simulink model "sschdlexTwoLevelConverterIdealModel"  (R2026a)
settings: Solver=FixedStepDiscrete  StopTime=20/fsw  MaxStep=1e-4  RelTol=1e-6  AbsTol=1e-6
InitFcn:
  | ts = 1e-5; % local solver sample period
  | fsw = 1e3; % switching frequency
libraries: nesl_utility x11, ee_lib x7, fl_lib x4, eePwmGeneratorTwoLevel x1
CloseFcn:
  | clear ts fsw;
settings Model: DataTypeOverride=Off  Creator=The MathWorks, Inc.  LastModifiedBy=The MathWorks, Inc.
settings DataIOCC: SaveFormat=StructureWithTime
settings OptimizationCC: ConditionallyExecuteInputs=off  OptimizeBlockIOStorage=off  BufferReuse=off  GlobalBufferReuse=off  ExpressionFolding=off  LocalBlockOutputs=off  OptimizeDataStoreBuffers=off  BusAssignmentInplaceUpdate=off
settings DebuggingCC: AlgebraicLoopMsg=error  SingleTaskRateTransMsg=error  PregeneratedLibrarySubsystemCodeDiagnostic=none
settings HardwareCC: ProdHWDeviceType=ASIC/FPGA->ASIC/FPGA  TargetBitPerLong=64.0  TargetBitPerPointer=64.0  TargetBitPerSizeT=64.0  TargetBitPerPtrDiffT=64.0  TargetLongLongMode=on  TargetIntDivRoundTo=Zero  TargetEndianess=LittleEndian  TargetWordSize=64.0  TargetHWDeviceType=Custom Processor->MATLAB Host Computer  ProdEqTarget=off
settings RTWCC: RTWCompilerOptimization=on
settings SimscapeCC: SimscapeNormalizeSystem=off  SimscapeNominalValues="[{\"value\":\"10\",\"unit\":\"V\"},{\"value\":\"1\",\"unit\":\"A\"},{\"value\":\"10\",\"unit\":\"N*m\"},{\"value\":\"10\",\"unit\":\"bar\"},{\"value\":\"100\",\"unit\":\"kJ/kg\"},{\"value\":\"1\",\"unit\":\"kW\"},{\"value\":\"300\",\"unit\":\"K\"},{\"value\":\"100\",\"unit\":\"cm^3/s\"},{\"value\":\"1\",\"unit\":\"kN\"},{\"value\":\"1\",\"unit\":\"g/cm^3\"},{\"value\":\"1\",\"unit\":\"l\"},{\"value\":\"1\",\"unit\":\"cm^2\"},{\"value\":\"60\",\"unit\":\"Hz\"}]"  SimscapeLogDataHistory=5000.0

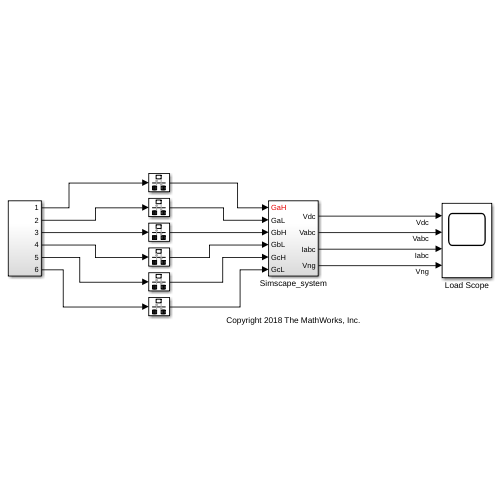
[thumbnail: Simulink's stored preview of the top-level diagram]
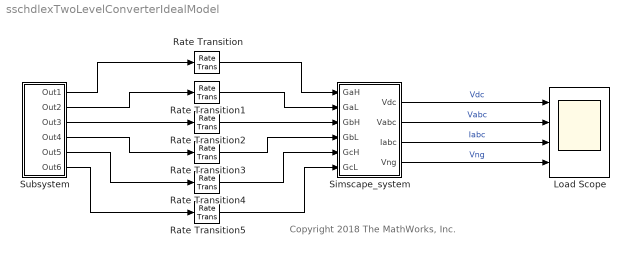
== system sschdlexTwoLevelConverterIdealModel ==
  note: Copyright 2018 The MathWorks, Inc.
  Load Scope : Scope  NumInputPorts=4
      settings: ActiveDisplayYMinimum=300  ActiveDisplayYMaximum=500  DataLoggingSaveFormat=Array
  Rate Transition{,1..5} (6 alike) : RateTransition
  Simscape_system : Subsystem
  Subsystem : Subsystem
  wires:
  Simscape_system/3(Iabc) -> Load Scope/3  "Iabc"
  Simscape_system/1(Vdc) -> Load Scope/1  "Vdc"
  Simscape_system/2(Vabc) -> Load Scope/2  "Vabc"
  Subsystem/1(Out1) -> Rate Transition/1
  Subsystem/2(Out2) -> Rate Transition1/1
  Subsystem/3(Out3) -> Rate Transition2/1
  Subsystem/4(Out4) -> Rate Transition3/1
  Subsystem/5(Out5) -> Rate Transition4/1
  Subsystem/6(Out6) -> Rate Transition5/1
  Rate Transition/1 -> Simscape_system/1(GaH)
  Rate Transition1/1 -> Simscape_system/2(GaL)
  Rate Transition2/1 -> Simscape_system/3(GbH)
  Rate Transition3/1 -> Simscape_system/4(GbL)
  Rate Transition4/1 -> Simscape_system/5(GcH)
  Rate Transition5/1 -> Simscape_system/6(GcL)
  Simscape_system/4(Vng) -> Load Scope/4  "Vng"

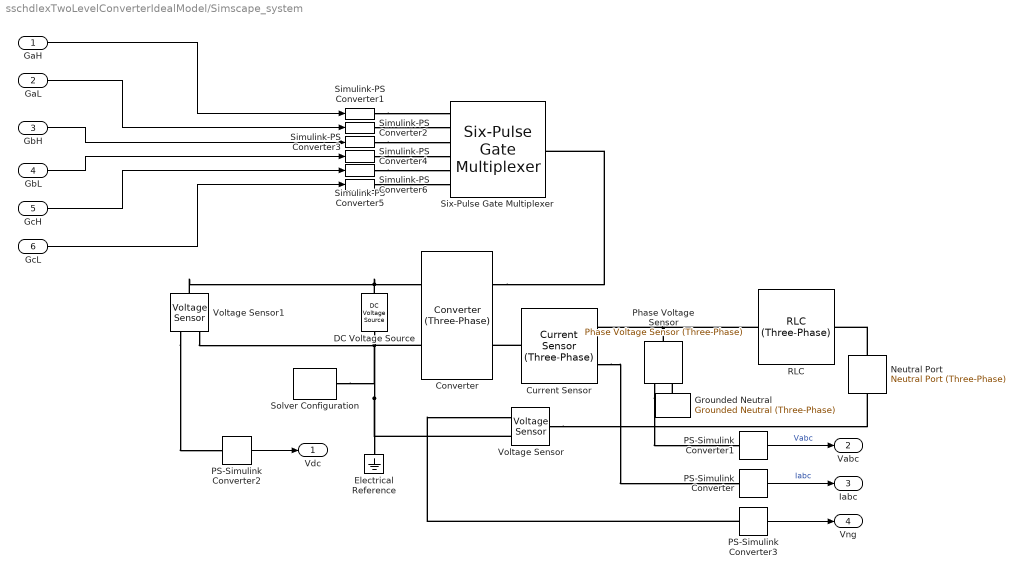
== system sschdlexTwoLevelConverterIdealModel/Simscape_system ==
  GaH : Inport
  GaL : Inport  Port=2
  GbH : Inport  Port=3
  GbL : Inport  Port=4
  GcH : Inport  Port=5
  GcL : Inport  Port=6
  Converter : ee_lib/Semiconductors & Converters/Converters/Converter (Three-Phase)  port_option=ee.enum.threePhasePort.composite  fidelity_option=ee.enum.converters.fidelity.detailed  device_type=2  showThermalPort=false  K=0  Vth=6 V  Vgt=1 V  Vgt_off=-1 V  Ih=1 A  Vf=0.8 V  Ron=0.001 Ohm  Rds=0.001 Ohm  Goff=1e-6 1/Ohm  Eon_scalar=22.86e-3 J  Eoff_scalar=17.14e-3 J  Eoff_natural_commutation=10e-3 J  Voff=300 V  Iout_scalar=600 A  onCurrentMeasDelay=0 s  useCurrentFromPreviousCycle=false  useVoltageFromPreviousCycle=false  diode_param=2  diode_Vf=0.8 V  diode_Ron=0.001 Ohm  diode_Goff=1e-5 1/Ohm  diode_C=50 nF  diode_iRM=-235 A  diode_iF=300 A  diode_idot=-50 A/us  diode_trr_param=1  diode_trr_factor=3  diode_trr=15 us  diode_Qrr=1.5e+3 s*uA  diode_rec_loss_model=ee.enum.diode.reverseRecoveryModel.fixed  diode_ErecVal=0 J  diode_scaleWithIandV=false  diode_ErecMat=zeros(2, 3) J  diode_TjrecVec=[298.15, 398.15] K  diode_IfrecVec=[.1, 1, 10] A  diode_IrecVal=10 A  diode_VrecVal=10 V  diode_tFilter=1 / 1000 / 100 s  thermal_network_parameterization=ee.enum.thermalNetworkTopology.external  Rth=[.08, .5] K/W  Rth_Cauer=[.08, .1, .5] K/W  Rth_Foster=[.08, .14, .22, .16] K/W  thermal_mass_parameterization=ee.enum.thermalNetwork.timeconstant  thermal_mass=[.01, .5] J/K  thermal_mass_Cauer=[.01, .1, .5] J/K  thermal_mass_Foster=[.001, .005, .05, .5] J/K  thermal_time_constant=[.001, .2] s  thermal_time_constant_Cauer=[.001, .1, .2] s  thermal_time_constant_Foster=[7e-05, .0007, .01, .08] s  thermal_mass_initial_temperatures=[25, 25] degC  thermal_mass_initial_temperatures_Cauer=[25, 25, 25] degC  junction_thermal_mass=0.01 J/K  Tvec_initial_Foster=[25, 25, 25, 25] degC  snubber_type=0  Cs=1e-7 F  Rs=0.1 Ohm  Vce_loss=[0, 150, 300] V
  Current Sensor : ee_lib/Sensors & Transducers/Current Sensor (Three-Phase)  port_option=ee.enum.threePhasePort.composite
  DC Voltage Source : fl_lib/Electrical/Electrical Sources/DC Voltage Source  v0=400 V
  Electrical Reference : fl_lib/Electrical/Electrical Elements/Electrical Reference
  Grounded Neutral : ee_lib/Connectors & References/Grounded Neutral (Three-Phase)  port_option=ee.enum.threePhasePort.composite
  Neutral Port : ee_lib/Connectors & References/Neutral Port (Three-Phase)  port_option=ee.enum.threePhasePort.composite  G_parasitic=1e-12 1/Ohm
  PS-Simulink Converter{,1..3} (4 alike) : nesl_utility/PS-Simulink Converter  PhysicalDomain=network_engine_domain  SubClassName=ps_output  LeftPortType=input  RightPortType=output  PseudoPeriodic=off  Frequencies=[]  VectorFormat=1-D array  Unit=1  AffineConversion=off
  Phase Voltage Sensor : ee_lib/Sensors & Transducers/Phase Voltage Sensor (Three-Phase)  port_option=ee.enum.threePhasePort.composite
  RLC : ee_lib/Passive/RLC Assemblies/RLC (Three-Phase)  port_option=ee.enum.threePhasePort.composite  component_structure=4  R=0.1 Ohm  L=0.001 H  C=1e-6 F  R_parasitic=1e-6 Ohm  G_parasitic=1e-6 1/Ohm  IL_specify=on  IL_priority=High  IL=[ 0 0 0 ] A  IL_nominal_specify=off  IL_nominal_value=1  IL_nominal_unit=A  VC_specify=on  VC_priority=High  VC=[ 0 0 0 ] V  VC_nominal_specify=off  VC_nominal_value=1  VC_nominal_unit=V
  Simulink-PS Converter{1..6} (6 alike) : nesl_utility/Simulink-PS Converter  PhysicalDomain=network_engine_domain  SubClassName=ps_input  LeftPortType=input  RightPortType=output  PseudoPeriodic=off  Frequencies=[]  NoiseDistribution=none  NoiseParameters=[]  Unit=1  AffineConversion=off  FilteringAndDerivatives=zero  SimscapeFilterOrder=1  InputFilterTimeConstant=0.001  UdotUserProvided=1
  Six-Pulse Gate Multiplexer : ee_lib/Semiconductors & Converters/Converters/Six-Pulse Gate Multiplexer  port_option=ee.enum.controlport.ps
  Solver Configuration : nesl_utility/Solver Configuration  PhysicalDomain=network_engine_domain  SubClassName=solver  LeftPortType=input  RightPortType=generic  Tones=[]  Harmonics=[]  SimulateNoise=off  Profile=off  UseLocalSampling=off  EnableSwitchedLinearOptims=on  FrequencyDomain=off  UseCCode=off  RelTol=0.001  AbsTol=1e-06  MinStep=1e-09  ToWorkspace=off  RevertToSquareIcSolve=off  NumHomotopyIterations=100  PhasorMode=off  PhasorModeNumHarmonics=1  ConsistencySolver=NEWTON_FTOL  CanonicalOrdering=UNORDERED  OptimizeIntermediates=UNOPTIMIZED  IndexReductionMethod=DerivativeReplacement  DoDC=off  ResidualTolerance=1e-09  ConsistencyTolSource=GLOBAL  ConsistencyAbsTol=0.001  ConsistencyRelTol=0.001  ConsistencyTolFactor=0.001  UseLocalSolver=on  LocalSolverChoice=NE_BACKWARD_EULER_ADVANCER  ResolveIndetEquations=on  FunctionEvalNumThread=1  LocalSolverSampleTime=ts  DoFixedCost=off  MaxNonlinIter=3  MaxModeIter=2  ComputeImpulses=off  ImpulseIterations=2  LinearAlgebra=Sparse  LinearAlgebraNumThread=0  EquationFormulation=NE_TIME_EF  DelaysMemoryBudget=1024  AutomaticFiltering=on  FilteringTimeConstant=0.001  PartitionStorageMethod=AS_NEEDED  PartitionMemoryBudget=1024  PartitionMethod=FAST  MultibodyUseLocalSolver=off  MultibodyLocalSolverChoice=ODE1  MultibodyLocalSolverSampleTime=0.001
  Voltage Sensor : fl_lib/Electrical/Electrical Sensors/Voltage Sensor
  Voltage Sensor1 : fl_lib/Electrical/Electrical Sensors/Voltage Sensor
  Vdc : Outport  VectorParamsAs1DForOutWhenUnconnected=off
  Vabc : Outport  Port=2  VectorParamsAs1DForOutWhenUnconnected=off
  Iabc : Outport  Port=3  VectorParamsAs1DForOutWhenUnconnected=off
  Vng : Outport  Port=4  VectorParamsAs1DForOutWhenUnconnected=off
  wires:
  PS-Simulink Converter2/1 -> Vdc/1
  PS-Simulink Converter/1 -> Iabc/1  "Iabc"
  GaH/1 -> Simulink-PS Converter1/1
  GbH/1 -> Simulink-PS Converter3/1
  GaL/1 -> Simulink-PS Converter2/1
  GbL/1 -> Simulink-PS Converter4/1
  GcH/1 -> Simulink-PS Converter5/1
  GcL/1 -> Simulink-PS Converter6/1
  PS-Simulink Converter1/1 -> Vabc/1  "Vabc"
  PS-Simulink Converter3/1 -> Vng/1
  connections:
  Current Sensor/LConn1 -- Converter/LConn2
  DC Voltage Source/LConn1 -- Voltage Sensor1/LConn1 -- Converter/RConn1
  Phase Voltage Sensor/RConn1 -- PS-Simulink Converter1/LConn1
  Simulink-PS Converter6/RConn1 -- Six-Pulse Gate Multiplexer/LConn6
  Simulink-PS Converter4/RConn1 -- Six-Pulse Gate Multiplexer/LConn4
  Simulink-PS Converter3/RConn1 -- Six-Pulse Gate Multiplexer/LConn3
  Simulink-PS Converter5/RConn1 -- Six-Pulse Gate Multiplexer/LConn5
  Converter/LConn1 -- Six-Pulse Gate Multiplexer/RConn1
  Simulink-PS Converter2/RConn1 -- Six-Pulse Gate Multiplexer/LConn2
  Simulink-PS Converter1/RConn1 -- Six-Pulse Gate Multiplexer/LConn1
  Voltage Sensor1/RConn1 -- PS-Simulink Converter2/LConn1
  Current Sensor/RConn1 -- PS-Simulink Converter/LConn1
  Phase Voltage Sensor/LConn1 -- RLC/LConn1 -- Current Sensor/RConn2
  Neutral Port/LConn1 -- RLC/RConn1
  Grounded Neutral/LConn1 -- Phase Voltage Sensor/RConn2
  Converter/RConn2 -- Solver Configuration/RConn1 -- Voltage Sensor/RConn2 -- Electrical Reference/LConn1 -- Voltage Sensor1/RConn2 -- DC Voltage Source/RConn1
  PS-Simulink Converter3/LConn1 -- Voltage Sensor/RConn1
  Voltage Sensor/LConn1 -- Neutral Port/RConn1

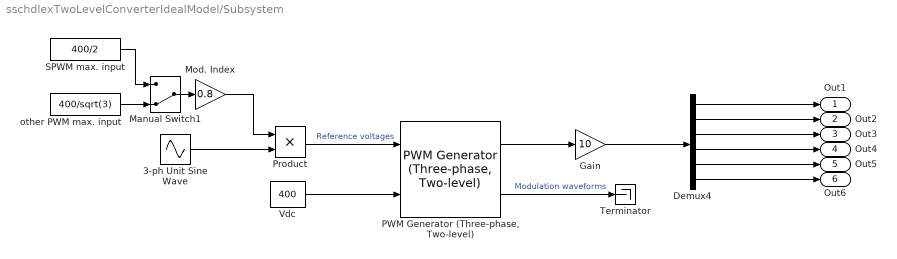
== system sschdlexTwoLevelConverterIdealModel/Subsystem ==
  3-ph Unit Sine Wave : Sin  Frequency=2*pi*60  Phase="[0  -2*pi/3  2*pi/3] + pi/2"  SampleTime=ts
  Demux4 : Demux  Outputs=6
  Gain : Gain  Gain=10
  Manual Switch1 : ManualSwitch  CurrentSetting=0
  Mod. Index : Gain  Gain=0.8
  "PWM Generator (Three-phase, Two-level)" : eePwmGeneratorTwoLevel/PWM Generator (Three-phase, Two-level)  PWMMode=Continuous PWM (CPWM)  CPWMMode=SVM: space vector modulation  DPWMMode=120 DPWM: positive dc component  fsw=fsw  Ts=ts
  Product : Product
  SPWM max. input : Constant  Value=400/2
  Terminator : Terminator
  Vdc : Constant  Value=400
  other PWM max. input : Constant  Value=400/sqrt(3)
  Out1 : Outport  VectorParamsAs1DForOutWhenUnconnected=off
  Out2 : Outport  Port=2  VectorParamsAs1DForOutWhenUnconnected=off
  Out3 : Outport  Port=3  VectorParamsAs1DForOutWhenUnconnected=off
  Out4 : Outport  Port=4  VectorParamsAs1DForOutWhenUnconnected=off
  Out5 : Outport  Port=5  VectorParamsAs1DForOutWhenUnconnected=off
  Out6 : Outport  Port=6  VectorParamsAs1DForOutWhenUnconnected=off
  wires:
  Gain/1 -> Demux4/1
  Demux4/6 -> Out6/1
  Demux4/1 -> Out1/1
  Demux4/3 -> Out3/1
  Demux4/5 -> Out5/1
  Demux4/4 -> Out4/1
  Demux4/2 -> Out2/1
  "PWM Generator (Three-phase, Two-level)"/1 -> Gain/1
  Product/1 -> "PWM Generator (Three-phase, Two-level)"/1  "Reference voltages"
  Vdc/1 -> "PWM Generator (Three-phase, Two-level)"/2
  other PWM max. input/1 -> Manual Switch1/2
  SPWM max. input/1 -> Manual Switch1/1
  Manual Switch1/1 -> Mod. Index/1
  "PWM Generator (Three-phase, Two-level)"/2 -> Terminator/1  "Modulation waveforms"
  Mod. Index/1 -> Product/1
  3-ph Unit Sine Wave/1 -> Product/2
